simulink model "PV_Station_Main"  (R2025a)
settings: Solver=ode45  StartTime=0.0  StopTime=86400  MaxStep=0.01  MinStep=1e-6  RelTol=1e-5  AbsTol=1e-8
libraries: simulink x1
settings Model: SimulationMode=accelerator  Creator=denis  LastModifiedBy=denis

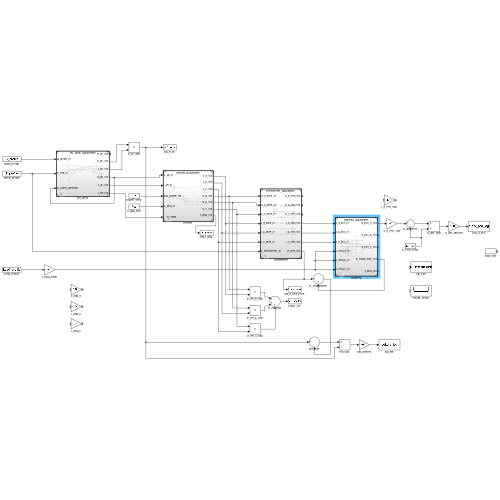
[thumbnail: Simulink's stored preview of the top-level diagram]
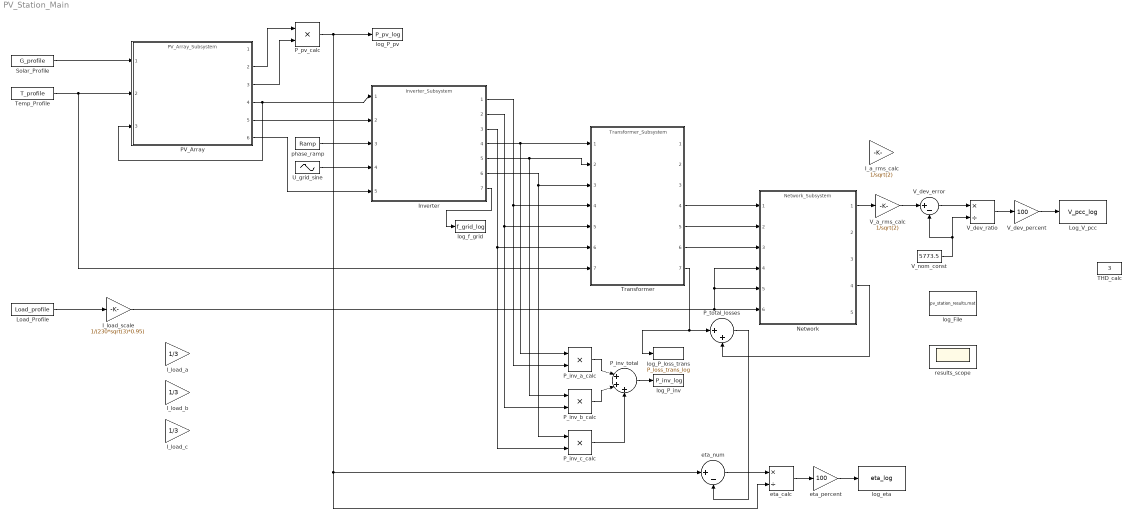
== system PV_Station_Main ==
  I_a_rms_calc : Gain  Gain=1/sqrt(2)
  I_load_a : Gain  Gain=1/3
  I_load_b : Gain  Gain=1/3
  I_load_c : Gain  Gain=1/3
  I_load_scale : Gain  Gain=1/(230*sqrt(3)*0.95)
  Inverter : ModelReference  ModelNameDialog=Inverter_Subsystem  SimulationMode=Normal  ModelReferenceVersion=1.1
  Load_Profile : FromWorkspace  VariableName=Load_profile  SampleTime=60
  Log_V_pcc : ToWorkspace  VariableName=V_pcc_log  SaveFormat=Structure With Time  SampleTime=-1
  Network : ModelReference  ModelNameDialog=Network_Subsystem  SimulationMode=Normal  ModelReferenceVersion=1.1
  PV_Array : ModelReference  ModelNameDialog=PV_Array_Subsystem  SimulationMode=Normal  ModelReferenceVersion=1.1
  P_inv_a_calc : Product
  P_inv_b_calc : Product
  P_inv_c_calc : Product
  P_inv_total : Sum  Inputs=|+++
  P_pv_calc : Product
  P_total_losses : Sum  Inputs=|++
  Solar_Profile : FromWorkspace  VariableName=G_profile  SampleTime=60
  THD_calc : Constant  Value=3
  Temp_Profile : FromWorkspace  VariableName=T_profile  SampleTime=60
  Transformer : ModelReference  ModelNameDialog=Transformer_Subsystem  SimulationMode=Normal  ModelReferenceVersion=1.1
  U_grid_sine : Sin  Amplitude=230  Frequency=50  SampleTime=0
  V_a_rms_calc : Gain  Gain=1/sqrt(2)
  V_dev_error : Sum  Inputs=|+-
  V_dev_percent : Gain  Gain=100
  V_dev_ratio : Product  Inputs=*/
  V_nom_const : Constant  Value=5773.5
  eta_calc : Product  Inputs=*/
  eta_num : Sum  Inputs=|+-
  eta_percent : Gain  Gain=100
  log_File : ToFile  Filename=pv_station_results.mat  SaveFormat=Timeseries
  log_P_inv : ToWorkspace  VariableName=P_inv_log  SampleTime=-1
  log_P_loss_trans : ToWorkspace  VariableName=P_loss_trans_log  SaveFormat=Structure With Time  SampleTime=-1
  log_P_pv : ToWorkspace  VariableName=P_pv_log  SampleTime=-1
  log_eta : ToWorkspace  VariableName=eta_log  SaveFormat=Structure With Time  SampleTime=-1
  log_f_grid : ToWorkspace  VariableName=f_grid_log  SampleTime=-1
  phase_ramp : simulink/Sources/Ramp  slope=314.159  start=0  InitialOutput=0
  results_scope : Scope
  wires:
  Solar_Profile/1 -> PV_Array/1
  Temp_Profile/1 -> PV_Array/2, Transformer/7
  PV_Array/4 -> Inverter/1, PV_Array/3
  PV_Array/2 -> P_pv_calc/1
  PV_Array/3 -> P_pv_calc/2
  P_pv_calc/1 -> eta_calc/2, eta_num/1, log_P_pv/1
  PV_Array/5 -> Inverter/2
  PV_Array/6 -> Inverter/5
  phase_ramp/1 -> Inverter/3
  U_grid_sine/1 -> Inverter/4
  Inverter/4 -> Transformer/1, P_inv_a_calc/1
  Inverter/5 -> Transformer/2, P_inv_b_calc/1
  Inverter/6 -> P_inv_c_calc/1, Transformer/3
  Inverter/1 -> P_inv_a_calc/2, Transformer/4
  Inverter/2 -> Transformer/5, P_inv_b_calc/2
  Inverter/3 -> P_inv_c_calc/2, Transformer/6
  Transformer/4 -> Network/1
  Transformer/5 -> Network/2
  Transformer/6 -> Network/3
  Load_Profile/1 -> I_load_scale/1
  I_load_scale/1 -> Network/4, Network/5, Network/6
  Network/1 -> V_a_rms_calc/1
  V_a_rms_calc/1 -> V_dev_error/1
  V_nom_const/1 -> V_dev_ratio/2, V_dev_error/2
  V_dev_error/1 -> V_dev_ratio/1
  V_dev_ratio/1 -> V_dev_percent/1
  V_dev_percent/1 -> Log_V_pcc/1
  Transformer/7 -> log_P_loss_trans/1, P_total_losses/1
  Inverter/7 -> log_f_grid/1
  Network/4 -> P_total_losses/2
  P_total_losses/1 -> eta_num/2
  eta_num/1 -> eta_calc/1
  eta_calc/1 -> eta_percent/1
  eta_percent/1 -> log_eta/1
  P_inv_a_calc/1 -> P_inv_total/1
  P_inv_b_calc/1 -> P_inv_total/2
  P_inv_c_calc/1 -> P_inv_total/3
  P_inv_total/1 -> log_P_inv/1
